simulink model "schema"  (R2023b)
settings: Solver=VariableStepAuto  StartTime=0.0  StopTime=10.0  RelTol=1e-3
settings Model: Creator=kseni  LastModifiedBy=kseni

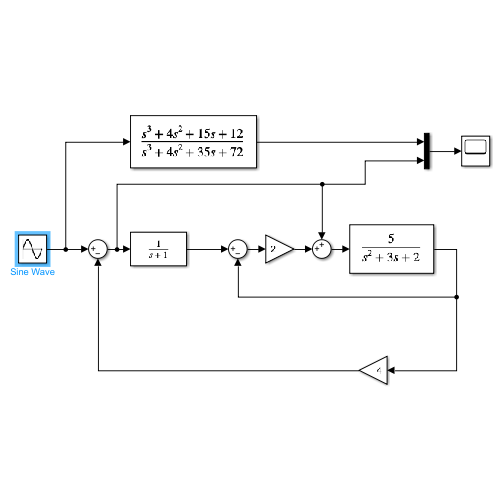
[thumbnail: Simulink's stored preview of the top-level diagram]
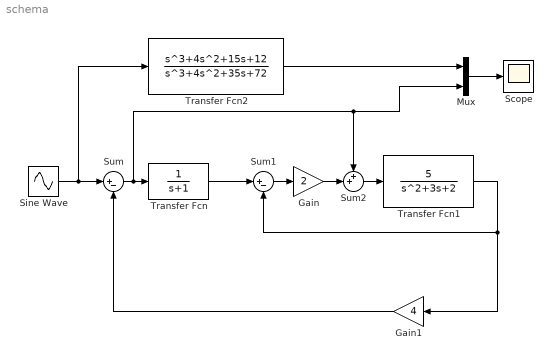
== system schema ==
  Gain : Gain  Gain=2
  Gain1 : Gain  Gain=4
  Mux : Mux  Inputs=2
  Scope : Scope
  Sine Wave : Sin  SampleTime=0
  Sum : Sum  Inputs=|+-
  Sum1 : Sum  Inputs=|+-
  Sum2 : Sum  Inputs=++|
  Transfer Fcn : TransferFcn  Denominator=[1 1]
  Transfer Fcn1 : TransferFcn  Numerator=[5]  Denominator=[1 3 2]
  Transfer Fcn2 : TransferFcn  Numerator=[1, 4, 15, 12]  Denominator=[1, 4, 35, 72]
  wires:
  Sum/1 -> Sum2/1, Mux/2, Transfer Fcn/1
  Transfer Fcn/1 -> Sum1/1
  Sum1/1 -> Gain/1
  Transfer Fcn1/1 -> Sum1/2, Gain1/1
  Gain1/1 -> Sum/2
  Gain/1 -> Sum2/2
  Sum2/1 -> Transfer Fcn1/1
  Sine Wave/1 -> Transfer Fcn2/1, Sum/1
  Transfer Fcn2/1 -> Mux/1
  Mux/1 -> Scope/1
